simulink model "A9_TCLab_MIL_CSD"  (R2026a)
settings: Solver=FixedStepDiscrete  StopTime=t_final  FixedStep=Ts
InitFcn:
  | A8_init_TCLab_SIMC
undefined symbols (not defined in the file): den_Gp_d, dspblkCoreblockFVToolHelper, gcbh, Ki_CSD, Ki_SIMC, Kp_CSD, Kp_SIMC, N_delay, num_Gp_d, Q_max, Q_min, T_amb, T_ref, Ts
libraries: slpidlib x2
settings Model: Creator=jguerrero  LastModifiedBy=jordy

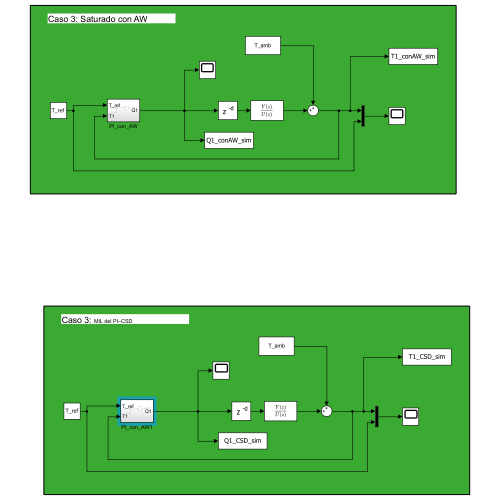
[thumbnail: Simulink's stored preview of the top-level diagram]
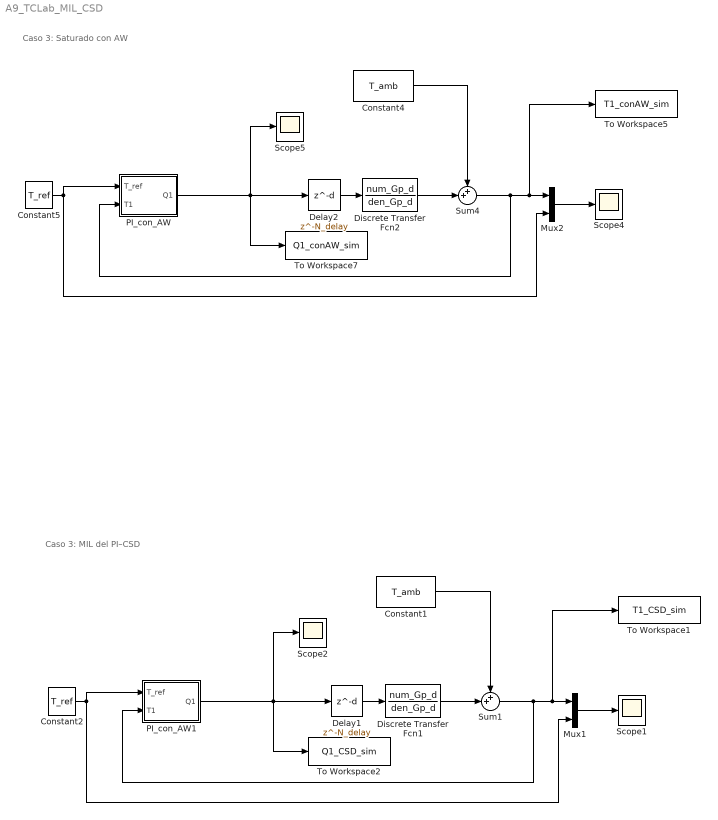
== system A9_TCLab_MIL_CSD ==
  note: Caso 3: Saturado con AW
  note: Caso 3: MIL del PI–CSD
  Constant1 : Constant  Value=T_amb
  Constant2 : Constant  Value=T_ref
  Constant4 : Constant  Value=T_amb
  Constant5 : Constant  Value=T_ref
  Delay1 : Delay  DelayLength=N_delay  SampleTime=Ts
  Delay2 : Delay  DelayLength=N_delay  SampleTime=Ts
  Discrete Transfer Fcn1 : DiscreteTransferFcn  LoadFcn=dspblkCoreblockFVToolHelper(gcbh,'load');  Numerator=num_Gp_d  Denominator=den_Gp_d
      settings: CopyFcn=dspblkCoreblockFVToolHelper(gcbh,'copy');  DeleteFcn=dspblkCoreblockFVToolHelper(gcbh,'close');  ModelCloseFcn=dspblkCoreblockFVToolHelper(gcbh,'close');  PreSaveFcn=dspblkCoreblockFVToolHelper(gcbh,'presave');  PostSaveFcn=dspblkCoreblockFVToolHelper(gcbh,'postsave');  CloseFcn=dspblkCoreblockFVToolHelper(gcbh,'close');
  Discrete Transfer Fcn2 : DiscreteTransferFcn  LoadFcn=dspblkCoreblockFVToolHelper(gcbh,'load');  Numerator=num_Gp_d  Denominator=den_Gp_d
      settings: CopyFcn=dspblkCoreblockFVToolHelper(gcbh,'copy');  DeleteFcn=dspblkCoreblockFVToolHelper(gcbh,'close');  ModelCloseFcn=dspblkCoreblockFVToolHelper(gcbh,'close');  PreSaveFcn=dspblkCoreblockFVToolHelper(gcbh,'presave');  PostSaveFcn=dspblkCoreblockFVToolHelper(gcbh,'postsave');  CloseFcn=dspblkCoreblockFVToolHelper(gcbh,'close');
  Mux1 : Mux  Inputs=2
  Mux2 : Mux  Inputs=2
  PI_con_AW : Subsystem
  PI_con_AW1 : Subsystem
  Scope{1..2,4..5} (4 alike) : Scope
      Scope1 settings: ActiveDisplayYMinimum=20.625  ActiveDisplayYMaximum=64.375
      Scope2 settings: ActiveDisplayYMinimum=27.921311930843586  ActiveDisplayYMaximum=96.897632007684052
      Scope4 settings: ActiveDisplayYMinimum=20.625  ActiveDisplayYMaximum=64.375  DataLoggingVariableName=ScopeData4
      Scope5 settings: ActiveDisplayYMinimum=27.921311930843586  ActiveDisplayYMaximum=96.897632007684052  DataLoggingVariableName=ScopeData5
  Sum1 : Sum  Inputs=++|
  Sum4 : Sum  Inputs=++|
  To Workspace1 : ToWorkspace  VariableName=T1_CSD_sim  SaveFormat=Timeseries  SampleTime=-1
  To Workspace2 : ToWorkspace  VariableName=Q1_CSD_sim  SaveFormat=Timeseries  SampleTime=-1
  To Workspace5 : ToWorkspace  VariableName=T1_conAW_sim  SaveFormat=Timeseries  SampleTime=-1
  To Workspace7 : ToWorkspace  VariableName=Q1_conAW_sim  SaveFormat=Timeseries  SampleTime=-1
  wires:
  Constant4/1 -> Sum4/1
  Sum4/1 -> PI_con_AW/2(T1), Mux2/1, To Workspace5/1
  Delay2/1 -> Discrete Transfer Fcn2/1
  Discrete Transfer Fcn2/1 -> Sum4/2
  Mux2/1 -> Scope4/1
  Constant5/1 -> PI_con_AW/1(T_ref), Mux2/2
  PI_con_AW/1(Q1) -> Scope5/1, To Workspace7/1, Delay2/1
  Discrete Transfer Fcn1/1 -> Sum1/2
  Sum1/1 -> PI_con_AW1/2(T1), Mux1/1, To Workspace1/1
  Delay1/1 -> Discrete Transfer Fcn1/1
  Mux1/1 -> Scope1/1
  Constant1/1 -> Sum1/1
  PI_con_AW1/1(Q1) -> Scope2/1, To Workspace2/1, Delay1/1
  Constant2/1 -> PI_con_AW1/1(T_ref), Mux1/2

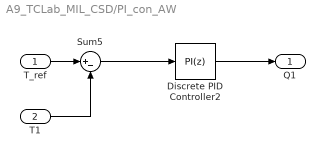
== system A9_TCLab_MIL_CSD/PI_con_AW ==
  T_ref : Inport
  T1 : Inport  Port=2
  Discrete PID Controller2 : slpidlib/PID Controller  Controller=PI  Form=Parallel  TimeDomain=Discrete-time  UseExternalTs=off  SampleTime=Ts  IntegratorMethod=Forward Euler  FilterMethod=Forward Euler  ControllerParametersSource=internal  P=Kp_SIMC  I=Ki_SIMC  UseKiTs=off  D=0  UseExternalDerivativeSource=off  N=100  UseFilter=on  TunerSelectOption=Transfer Function Based (PID Tuner App)  InitialConditionSource=internal  InitialConditionForIntegrator=0  InitialConditionForFilter=0  DifferentiatorICPrevScaledInput=0  ExternalReset=none  TrackingMode=off  Kt=1  LimitOutput=on  SatLimitsSource=internal  UpperSaturationLimit=Q_max  LowerSaturationLimit=Q_min  LinearizeAsGain=off  AntiWindupMode=clamping  Kb=1  LimitIntegrator=off  UpperIntegratorSaturationLimit=inf  LowerIntegratorSaturationLimit=-inf  POutMin=[]  POutMax=[]  IOutMin=[]  IOutMax=[]  DOutMin=[]  DOutMax=[]  NOutMin=[]  NOutMax=[]  SumOutMin=[]  SumOutMax=[]  SaturationOutMin=[]  SaturationOutMax=[]  PParamMin=[]  PParamMax=[]  IParamMin=[]  IParamMax=[]  DParamMin=[]  DParamMax=[]  NParamMin=[]  NParamMax=[]  KbParamMin=[]  KbParamMax=[]  KtParamMin=[]  KtParamMax=[]  KbOutMin=[]  KbOutMax=[]  KtOutMin=[]  KtOutMax=[]  IntegratorOutMin=[]  IntegratorOutMax=[]  FilterOutMin=[]  FilterOutMax=[]  SumI1OutMin=[]  SumI1OutMax=[]  SumI2OutMin=[]  SumI2OutMax=[]  SumI3OutMin=[]  SumI3OutMax=[]  SumI4OutMin=[]  SumI4OutMax=[]  SumDOutMin=[]  SumDOutMax=[]  DifferentiatorOutMin=[]  DifferentiatorOutMax=[]  FilterDiffOutCoefMin=[]  FilterDiffOutCoefMax=[]  ReciprocalOutMin=[]  ReciprocalOutMax=[]  SumDenOutMin=[]  SumDenOutMax=[]  SumNumOutMin=[]  SumNumOutMax=[]  DivideOutMin=[]  DivideOutMax=[]  UdiffTsProdOutMin=[]  UdiffTsProdOutMax=[]  NTsProdOutMin=[]  NTsProdOutMax=[]  UintegralTsProdOutMin=[]  UintegralTsProdOutMax=[]  UngainTsProdOutMin=[]  UngainTsProdOutMax=[]  ClampingZeroOutDataTypeStr=Inherit: Inherit via back propagation  ClampingZeroOutMin=[]  ClampingZeroOutMax=[]  FilterDenConstantOutDataTypeStr=Inherit: Inherit via back propagation  FilterDenConstantOutMin=[]  FilterDenConstantOutMax=[]  PCopyOutDataTypeStr=Inherit: Inherit via back propagation  PCopyOutMin=[]  PCopyOutMax=[]  NCopyOutDataTypeStr=Inherit: Inherit via back propagation  NCopyOutMin=[]  NCopyOutMax=[]  IntegratorContinuousStateAttributes=''  IntegratorStateMustResolveToSignalObject=off  IntegratorRTWStateStorageClass=Auto  FilterContinuousStateAttributes=''  FilterStateMustResolveToSignalObject=off  FilterRTWStateStorageClass=Auto  ParallelPVariant=InternalParameters  IdealPVariant=Disabled  IVariant=InternalParameters  DVariant=Disabled  IntegratorVariant=Discrete  SatVariant=Enabled  AWVariant=DiscClampingParallel  PCopyVariant=Disabled  TRVariant=Disabled  FdbkBlocksVariant=Forward  IdealPFdbkVariant=Disabled  SatFdbkVariant=Disabled  DerivativeFilterVariant=Disabled  NVariant=Disabled  NCopyVariant=Disabled_SignalSpec  FilterICVariant=Disabled  IntegratorICVariant=InternalICs  ExternalResetVariant=Disabled  TRSumVariant=Passthrough  SumFdbkVariant=Disabled  SumVariant=Sum_PI  TsampFilterVariant=InternalTs  TsampNgainVariant=Passthrough  TsampIntegralVariant=Disabled_SignalSpec  ExternalSaturationOutDataTypeStr=Inherit: Same as second input  DerivativeSourceVariant=Disabled  PreIntVariant=InternalPreInt
      settings: LibrarySourceBlock=simulink/Discrete/Discrete PID Controller
  Sum5 : Sum  Inputs=|+-
  Q1 : Outport
  wires:
  Sum5/1 -> Discrete PID Controller2/1
  T_ref/1 -> Sum5/1
  T1/1 -> Sum5/2
  Discrete PID Controller2/1 -> Q1/1

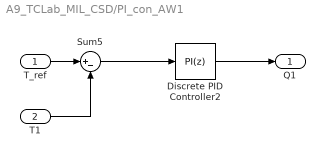
== system A9_TCLab_MIL_CSD/PI_con_AW1 ==
  T_ref : Inport
  T1 : Inport  Port=2
  Discrete PID Controller2 : slpidlib/PID Controller  Controller=PI  Form=Parallel  TimeDomain=Discrete-time  UseExternalTs=off  SampleTime=Ts  IntegratorMethod=Forward Euler  FilterMethod=Forward Euler  ControllerParametersSource=internal  P=Kp_CSD  I=Ki_CSD  UseKiTs=off  D=0  UseExternalDerivativeSource=off  N=100  UseFilter=on  TunerSelectOption=Transfer Function Based (PID Tuner App)  InitialConditionSource=internal  InitialConditionForIntegrator=0  InitialConditionForFilter=0  DifferentiatorICPrevScaledInput=0  ExternalReset=none  TrackingMode=off  Kt=1  LimitOutput=on  SatLimitsSource=internal  UpperSaturationLimit=Q_max  LowerSaturationLimit=Q_min  LinearizeAsGain=off  AntiWindupMode=clamping  Kb=1  LimitIntegrator=off  UpperIntegratorSaturationLimit=inf  LowerIntegratorSaturationLimit=-inf  POutMin=[]  POutMax=[]  IOutMin=[]  IOutMax=[]  DOutMin=[]  DOutMax=[]  NOutMin=[]  NOutMax=[]  SumOutMin=[]  SumOutMax=[]  SaturationOutMin=[]  SaturationOutMax=[]  PParamMin=[]  PParamMax=[]  IParamMin=[]  IParamMax=[]  DParamMin=[]  DParamMax=[]  NParamMin=[]  NParamMax=[]  KbParamMin=[]  KbParamMax=[]  KtParamMin=[]  KtParamMax=[]  KbOutMin=[]  KbOutMax=[]  KtOutMin=[]  KtOutMax=[]  IntegratorOutMin=[]  IntegratorOutMax=[]  FilterOutMin=[]  FilterOutMax=[]  SumI1OutMin=[]  SumI1OutMax=[]  SumI2OutMin=[]  SumI2OutMax=[]  SumI3OutMin=[]  SumI3OutMax=[]  SumI4OutMin=[]  SumI4OutMax=[]  SumDOutMin=[]  SumDOutMax=[]  DifferentiatorOutMin=[]  DifferentiatorOutMax=[]  FilterDiffOutCoefMin=[]  FilterDiffOutCoefMax=[]  ReciprocalOutMin=[]  ReciprocalOutMax=[]  SumDenOutMin=[]  SumDenOutMax=[]  SumNumOutMin=[]  SumNumOutMax=[]  DivideOutMin=[]  DivideOutMax=[]  UdiffTsProdOutMin=[]  UdiffTsProdOutMax=[]  NTsProdOutMin=[]  NTsProdOutMax=[]  UintegralTsProdOutMin=[]  UintegralTsProdOutMax=[]  UngainTsProdOutMin=[]  UngainTsProdOutMax=[]  ClampingZeroOutDataTypeStr=Inherit: Inherit via back propagation  ClampingZeroOutMin=[]  ClampingZeroOutMax=[]  FilterDenConstantOutDataTypeStr=Inherit: Inherit via back propagation  FilterDenConstantOutMin=[]  FilterDenConstantOutMax=[]  PCopyOutDataTypeStr=Inherit: Inherit via back propagation  PCopyOutMin=[]  PCopyOutMax=[]  NCopyOutDataTypeStr=Inherit: Inherit via back propagation  NCopyOutMin=[]  NCopyOutMax=[]  IntegratorContinuousStateAttributes=''  IntegratorStateMustResolveToSignalObject=off  IntegratorRTWStateStorageClass=Auto  FilterContinuousStateAttributes=''  FilterStateMustResolveToSignalObject=off  FilterRTWStateStorageClass=Auto  ParallelPVariant=InternalParameters  IdealPVariant=Disabled  IVariant=InternalParameters  DVariant=Disabled  IntegratorVariant=Discrete  SatVariant=Enabled  AWVariant=DiscClampingParallel  PCopyVariant=Disabled  TRVariant=Disabled  FdbkBlocksVariant=Forward  IdealPFdbkVariant=Disabled  SatFdbkVariant=Disabled  DerivativeFilterVariant=Disabled  NVariant=Disabled  NCopyVariant=Disabled_SignalSpec  FilterICVariant=Disabled  IntegratorICVariant=InternalICs  ExternalResetVariant=Disabled  TRSumVariant=Passthrough  SumFdbkVariant=Disabled  SumVariant=Sum_PI  TsampFilterVariant=InternalTs  TsampNgainVariant=Passthrough  TsampIntegralVariant=Disabled_SignalSpec  ExternalSaturationOutDataTypeStr=Inherit: Same as second input  DerivativeSourceVariant=Disabled  PreIntVariant=InternalPreInt
      settings: LibrarySourceBlock=simulink/Discrete/Discrete PID Controller
  Sum5 : Sum  Inputs=|+-
  Q1 : Outport
  wires:
  Sum5/1 -> Discrete PID Controller2/1
  T_ref/1 -> Sum5/1
  T1/1 -> Sum5/2
  Discrete PID Controller2/1 -> Q1/1
